simulink model "rfsoc4x2_ospfb_128"  (R2021a)
settings: Solver=VariableStepAuto  StartTime=0.0  StopTime=2048  RelTol=1e-3
undefined symbols (not defined in the file): pfb_coeff_gen_calc
libraries: xbsIndex_r4 x37092, casper_library_delays x737, casper_library_misc x68, xps_library x1
(part 157 of 339)

== system rfsoc4x2_ospfb_128/fft_wideband_real1/fft_unscrambler/reorder ==
  sync : Inport
  en : Inport  Port=2
  din0 : Inport  Port=3
  din1 : Inport  Port=4
  din2 : Inport  Port=5
  din3 : Inport  Port=6
  din4 : Inport  Port=7
  din5 : Inport  Port=8
  din6 : Inport  Port=9
  din7 : Inport  Port=10
  Counter : xbsIndex_r4/Counter  cnt_type=Free Running  cnt_to=Inf  operation=Up  start_count=0  cnt_by_val=1  arith_type=Unsigned  n_bits=4  bin_pt=0  load_pin=off  rst=on  en=on  explicit_period=on  period=1  use_behavioral_HDL=on  implementation=Fabric  dbl_ovrd=off  block_type=counter
  addr_expand : Subsystem  AncestorBlock=casper_library_flow_control/bus_expand  mask(bus_expand){mode=divisions of equal size, outputNum=8, outputWidth=4, outputBinaryPt=0, outputArithmeticType=0, show_format=off, outputToWorkspace=off, variablePrefix=out, outputToModelAsWell=on}
      mask prompts: outputNum "Number of outputs:"; outputWidth "Output width:"; outputBinaryPt "Output binary point position:"; outputArithmeticType "Output arithmetic type (ufix=0, fix=1, bool=2):"; show_format "Print format string?"; outputToWorkspace "Output to workspace?"; variablePrefix "Variable name prefix:"; outputToModelAsWell "Output to model as well?"
      mask help:
      | Expands a 'bus' made using a bus_create or Xilinx
      | concat block.
      | The input will be divided into the specified number
      | of outputs with the specified arithmetic types.
      | Divisions are made from most significant bit.
      mask init: same as rfsoc4x2_ospfb_128/bus_expand1
      settings: AttributesFormatString=8 outputs
      mask TypeOptions mode: divisions of equal size | divisions of arbitrary size
      mask Callback mode: %bus_expand_callback();
      mask Callback outputWidth: %bus_expand_callback();
      mask Callback outputToWorkspace: %bus_expand_callback();
  addr_replicate : Subsystem  AncestorBlock=casper_library_bus/bus_replicate  mask(bus_replicate){replication=8, csp_latency=3, misc=off, implementation=core}
      mask prompts: replication "replication factor"; csp_latency "latency"; misc "misc support"; implementation "delay implementation"
      mask help: Output bus formed by replicating input bus a number of times
      mask init:
      | bus_replicate_init(gcb, ...
      |     'replication', replication, ...
      |     'csp_latency', csp_latency, ...
      |     'implementation', implementation, ...
      |     'misc', misc);
      mask TypeOptions implementation: core | behavioral
  blank : xbsIndex_r4/Constant  const=0  gui_display_data_type=Fixed-point  arith_type=Unsigned  n_bits=4  bin_pt=0  preci_type=Single  exp_width=8  frac_width=24  explicit_period=on  period=1  equ=P=C  opselect=C  inp2=PCIN>>17  opr=+  inp1=P  carry=CIN  dbl_ovrd=off  block_type=constant
  buf0 : Subsystem  AncestorBlock=casper_library_bus/bus_single_port_ram  mask(bus_single_port_ram){n_bits=[[repmat(64, 1, 0)], 36], bin_pts=[zeros(1, 1)], init_vector=[zeros(16,1)], max_fanout=1, mem_type=Block RAM, bram_optimization=Speed, async=off, misc=off, bram_latency=3, fan_latency=0, addr_register=on, addr_implementation=core, din_register=on, din_implementation=behavioral, we_register=on, we_implementation=core, en_register=off, en_implementation=behavioral}
      mask prompts: n_bits "data word bit widths"; bin_pts "data word binary points"; init_vector "initial value vector"; max_fanout "limit fanout to ?"; mem_type "memory type"; bram_optimization "memory optimization"; async "asynchronous"; misc "misc support"; bram_latency "bram latency"; fan_latency "input register latency"; addr_register "addr input register"; addr_implementation "addr register implementation"; din_register "din input register"; din_implementation "din register implementation"; we_register "we input register"; we_implementation "we register implementation"; en_register "en input register"; en_implementation "en register implementation"
      mask help: RAM for a bus allowing fanout control
      mask init: same as rfsoc4x2_ospfb_128/fft2/fft_unscrambler/reorder/buf0
      mask TypeOptions mem_type: Distributed memory | Block RAM
      mask TypeOptions bram_optimization: Area | Speed
      mask TypeOptions addr_implementation: core | behavioral
      mask TypeOptions din_implementation: core | behavioral
      mask TypeOptions we_implementation: core | behavioral
      mask TypeOptions en_implementation: core | behavioral
  buf1 : Subsystem  AncestorBlock=casper_library_bus/bus_single_port_ram  mask(bus_single_port_ram){n_bits=[[repmat(64, 1, 0)], 36], bin_pts=[zeros(1, 1)], init_vector=[zeros(16,1)], max_fanout=1, mem_type=Block RAM, bram_optimization=Speed, async=off, misc=off, bram_latency=3, fan_latency=0, addr_register=on, addr_implementation=core, din_register=on, din_implementation=behavioral, we_register=on, we_implementation=core, en_register=off, en_implementation=behavioral}
      mask prompts: n_bits "data word bit widths"; bin_pts "data word binary points"; init_vector "initial value vector"; max_fanout "limit fanout to ?"; mem_type "memory type"; bram_optimization "memory optimization"; async "asynchronous"; misc "misc support"; bram_latency "bram latency"; fan_latency "input register latency"; addr_register "addr input register"; addr_implementation "addr register implementation"; din_register "din input register"; din_implementation "din register implementation"; we_register "we input register"; we_implementation "we register implementation"; en_register "en input register"; en_implementation "en register implementation"
      mask help: RAM for a bus allowing fanout control
      mask init: same as rfsoc4x2_ospfb_128/fft2/fft_unscrambler/reorder/buf0
      mask TypeOptions mem_type: Distributed memory | Block RAM
      mask TypeOptions bram_optimization: Area | Speed
      mask TypeOptions addr_implementation: core | behavioral
      mask TypeOptions din_implementation: core | behavioral
      mask TypeOptions we_implementation: core | behavioral
      mask TypeOptions en_implementation: core | behavioral
  buf2 : Subsystem  AncestorBlock=casper_library_bus/bus_single_port_ram  mask(bus_single_port_ram){n_bits=[[repmat(64, 1, 0)], 36], bin_pts=[zeros(1, 1)], init_vector=[zeros(16,1)], max_fanout=1, mem_type=Block RAM, bram_optimization=Speed, async=off, misc=off, bram_latency=3, fan_latency=0, addr_register=on, addr_implementation=core, din_register=on, din_implementation=behavioral, we_register=on, we_implementation=core, en_register=off, en_implementation=behavioral}
      mask prompts: n_bits "data word bit widths"; bin_pts "data word binary points"; init_vector "initial value vector"; max_fanout "limit fanout to ?"; mem_type "memory type"; bram_optimization "memory optimization"; async "asynchronous"; misc "misc support"; bram_latency "bram latency"; fan_latency "input register latency"; addr_register "addr input register"; addr_implementation "addr register implementation"; din_register "din input register"; din_implementation "din register implementation"; we_register "we input register"; we_implementation "we register implementation"; en_register "en input register"; en_implementation "en register implementation"
      mask help: RAM for a bus allowing fanout control
      mask init: same as rfsoc4x2_ospfb_128/fft2/fft_unscrambler/reorder/buf0
      mask TypeOptions mem_type: Distributed memory | Block RAM
      mask TypeOptions bram_optimization: Area | Speed
      mask TypeOptions addr_implementation: core | behavioral
      mask TypeOptions din_implementation: core | behavioral
      mask TypeOptions we_implementation: core | behavioral
      mask TypeOptions en_implementation: core | behavioral
  buf3 : Subsystem  AncestorBlock=casper_library_bus/bus_single_port_ram  mask(bus_single_port_ram){n_bits=[[repmat(64, 1, 0)], 36], bin_pts=[zeros(1, 1)], init_vector=[zeros(16,1)], max_fanout=1, mem_type=Block RAM, bram_optimization=Speed, async=off, misc=off, bram_latency=3, fan_latency=0, addr_register=on, addr_implementation=core, din_register=on, din_implementation=behavioral, we_register=on, we_implementation=core, en_register=off, en_implementation=behavioral}
      mask prompts: n_bits "data word bit widths"; bin_pts "data word binary points"; init_vector "initial value vector"; max_fanout "limit fanout to ?"; mem_type "memory type"; bram_optimization "memory optimization"; async "asynchronous"; misc "misc support"; bram_latency "bram latency"; fan_latency "input register latency"; addr_register "addr input register"; addr_implementation "addr register implementation"; din_register "din input register"; din_implementation "din register implementation"; we_register "we input register"; we_implementation "we register implementation"; en_register "en input register"; en_implementation "en register implementation"
      mask help: RAM for a bus allowing fanout control
      mask init: same as rfsoc4x2_ospfb_128/fft2/fft_unscrambler/reorder/buf0
      mask TypeOptions mem_type: Distributed memory | Block RAM
      mask TypeOptions bram_optimization: Area | Speed
      mask TypeOptions addr_implementation: core | behavioral
      mask TypeOptions din_implementation: core | behavioral
      mask TypeOptions we_implementation: core | behavioral
      mask TypeOptions en_implementation: core | behavioral
  buf4 : Subsystem  AncestorBlock=casper_library_bus/bus_single_port_ram  mask(bus_single_port_ram){n_bits=[[repmat(64, 1, 0)], 36], bin_pts=[zeros(1, 1)], init_vector=[zeros(16,1)], max_fanout=1, mem_type=Block RAM, bram_optimization=Speed, async=off, misc=off, bram_latency=3, fan_latency=0, addr_register=on, addr_implementation=core, din_register=on, din_implementation=behavioral, we_register=on, we_implementation=core, en_register=off, en_implementation=behavioral}
      mask prompts: n_bits "data word bit widths"; bin_pts "data word binary points"; init_vector "initial value vector"; max_fanout "limit fanout to ?"; mem_type "memory type"; bram_optimization "memory optimization"; async "asynchronous"; misc "misc support"; bram_latency "bram latency"; fan_latency "input register latency"; addr_register "addr input register"; addr_implementation "addr register implementation"; din_register "din input register"; din_implementation "din register implementation"; we_register "we input register"; we_implementation "we register implementation"; en_register "en input register"; en_implementation "en register implementation"
      mask help: RAM for a bus allowing fanout control
      mask init: same as rfsoc4x2_ospfb_128/fft2/fft_unscrambler/reorder/buf0
      mask TypeOptions mem_type: Distributed memory | Block RAM
      mask TypeOptions bram_optimization: Area | Speed
      mask TypeOptions addr_implementation: core | behavioral
      mask TypeOptions din_implementation: core | behavioral
      mask TypeOptions we_implementation: core | behavioral
      mask TypeOptions en_implementation: core | behavioral
  buf5 : Subsystem  AncestorBlock=casper_library_bus/bus_single_port_ram  mask(bus_single_port_ram){n_bits=[[repmat(64, 1, 0)], 36], bin_pts=[zeros(1, 1)], init_vector=[zeros(16,1)], max_fanout=1, mem_type=Block RAM, bram_optimization=Speed, async=off, misc=off, bram_latency=3, fan_latency=0, addr_register=on, addr_implementation=core, din_register=on, din_implementation=behavioral, we_register=on, we_implementation=core, en_register=off, en_implementation=behavioral}
      mask prompts: n_bits "data word bit widths"; bin_pts "data word binary points"; init_vector "initial value vector"; max_fanout "limit fanout to ?"; mem_type "memory type"; bram_optimization "memory optimization"; async "asynchronous"; misc "misc support"; bram_latency "bram latency"; fan_latency "input register latency"; addr_register "addr input register"; addr_implementation "addr register implementation"; din_register "din input register"; din_implementation "din register implementation"; we_register "we input register"; we_implementation "we register implementation"; en_register "en input register"; en_implementation "en register implementation"
      mask help: RAM for a bus allowing fanout control
      mask init: same as rfsoc4x2_ospfb_128/fft2/fft_unscrambler/reorder/buf0
      mask TypeOptions mem_type: Distributed memory | Block RAM
      mask TypeOptions bram_optimization: Area | Speed
      mask TypeOptions addr_implementation: core | behavioral
      mask TypeOptions din_implementation: core | behavioral
      mask TypeOptions we_implementation: core | behavioral
      mask TypeOptions en_implementation: core | behavioral
  buf6 : Subsystem  AncestorBlock=casper_library_bus/bus_single_port_ram  mask(bus_single_port_ram){n_bits=[[repmat(64, 1, 0)], 36], bin_pts=[zeros(1, 1)], init_vector=[zeros(16,1)], max_fanout=1, mem_type=Block RAM, bram_optimization=Speed, async=off, misc=off, bram_latency=3, fan_latency=0, addr_register=on, addr_implementation=core, din_register=on, din_implementation=behavioral, we_register=on, we_implementation=core, en_register=off, en_implementation=behavioral}
      mask prompts: n_bits "data word bit widths"; bin_pts "data word binary points"; init_vector "initial value vector"; max_fanout "limit fanout to ?"; mem_type "memory type"; bram_optimization "memory optimization"; async "asynchronous"; misc "misc support"; bram_latency "bram latency"; fan_latency "input register latency"; addr_register "addr input register"; addr_implementation "addr register implementation"; din_register "din input register"; din_implementation "din register implementation"; we_register "we input register"; we_implementation "we register implementation"; en_register "en input register"; en_implementation "en register implementation"
      mask help: RAM for a bus allowing fanout control
      mask init: same as rfsoc4x2_ospfb_128/fft2/fft_unscrambler/reorder/buf0
      mask TypeOptions mem_type: Distributed memory | Block RAM
      mask TypeOptions bram_optimization: Area | Speed
      mask TypeOptions addr_implementation: core | behavioral
      mask TypeOptions din_implementation: core | behavioral
      mask TypeOptions we_implementation: core | behavioral
      mask TypeOptions en_implementation: core | behavioral
  buf7 : Subsystem  AncestorBlock=casper_library_bus/bus_single_port_ram  mask(bus_single_port_ram){n_bits=[[repmat(64, 1, 0)], 36], bin_pts=[zeros(1, 1)], init_vector=[zeros(16,1)], max_fanout=1, mem_type=Block RAM, bram_optimization=Speed, async=off, misc=off, bram_latency=3, fan_latency=0, addr_register=on, addr_implementation=core, din_register=on, din_implementation=behavioral, we_register=on, we_implementation=core, en_register=off, en_implementation=behavioral}
      mask prompts: n_bits "data word bit widths"; bin_pts "data word binary points"; init_vector "initial value vector"; max_fanout "limit fanout to ?"; mem_type "memory type"; bram_optimization "memory optimization"; async "asynchronous"; misc "misc support"; bram_latency "bram latency"; fan_latency "input register latency"; addr_register "addr input register"; addr_implementation "addr register implementation"; din_register "din input register"; din_implementation "din register implementation"; we_register "we input register"; we_implementation "we register implementation"; en_register "en input register"; en_implementation "en register implementation"
      mask help: RAM for a bus allowing fanout control
      mask init: same as rfsoc4x2_ospfb_128/fft2/fft_unscrambler/reorder/buf0
      mask TypeOptions mem_type: Distributed memory | Block RAM
      mask TypeOptions bram_optimization: Area | Speed
      mask TypeOptions addr_implementation: core | behavioral
      mask TypeOptions din_implementation: core | behavioral
      mask TypeOptions we_implementation: core | behavioral
      mask TypeOptions en_implementation: core | behavioral
  current_map : Subsystem  AncestorBlock=casper_library_bus/bus_dual_port_ram  mask(bus_dual_port_ram){n_bits=4, bin_pts=0, init_vector=[0:15]', max_fanout=1, mem_type=Block RAM, bram_optimization=Speed, async_a=off, async_b=off, b_to_a_ratio_bits=0, misc=off, bram_latency=2, fan_latency=4, addra_register=on, addra_implementation=behavioral, dina_register=off, dina_implementation=behavioral, wea_register=on, wea_implementation=core, ena_register=off, ena_implementation=core, addrb_register=off, addrb_implementation=core, dinb_register=off, dinb_implementation=behavioral, web_register=off, web_implementation=behavioral, enb_register=off, enb_implementation=core}
      mask prompts: n_bits "data word bit widths"; bin_pts "data word binary points"; init_vector "initial value vector"; max_fanout "limit fanout to ?"; mem_type "memory type"; bram_optimization "memory optimization"; async_a "a asynchronous"; async_b "b asynchronous"; b_to_a_ratio_bits "b_to_a ratio bits"; misc "misc support"; bram_latency "bram latency"; fan_latency "input register latency"; addra_register "addra input register"; addra_implementation "addra register implementation"; dina_register "dina input register"; dina_implementation "dina register implementation"; wea_register "wea input register"; wea_implementation "wea register implementation"; ena_register "ena input register"; ena_implementation "ena register implementation"; addrb_register "addrb input register"; addrb_implementation "addrb register implementation"; dinb_register "dinb input register"; dinb_implementation "dinb register implementation"; web_register "web input register"; web_implementation "web register implementation"; enb_register "enb input register"; enb_implementation "enb register implementation"
      mask help: RAM for a bus allowing fanout control
      mask init:
      | bus_dual_port_ram_init(gcb, ...
      |     'n_bits', n_bits, ...
      |     'bin_pts', bin_pts, ...
      |     'init_vector', init_vector, ...
      |     'max_fanout', max_fanout, ...
      |     'mem_type', mem_type, ...
      |     'bram_optimization', bram_optimization, ...
      |     'async_a', async_a, ...
      |     'async_b', async_b, ...
      |     'b_to_a_ratio_bits', b_to_a_ratio_bits, ...
      |     'misc', misc, ...
      |     'bram_latency', bram_latency, ...
      |     'fan_latency', fan_latency, ...
      |     'addra_register', addra_register, ...
      |     'addra_implementation', addra_implementation, ...
      |     'dina_register', dina_register, ...
      |     'dina_implementation', dina_implementation, ...
      |     'wea_register', wea_register, ...
      |     'wea_implementation', wea_implementation, ...
      |     'ena_register', ena_register, ...
      |     'ena_implementation', ena_implementation, ...
      |     'addrb_register', addrb_register, ...
      |     'addrb_implementation', addrb_implementation, ...
      |     'dinb_register', dinb_register, ...
      |     'dinb_implementation', dinb_implementation, ...
      |     'web_register', web_register, ...
      |     'web_implementation', web_implementation, ...
      |     'enb_register', enb_register, ...
      |     'enb_implementation', enb_implementation);
      mask TypeOptions mem_type: Distributed memory | Block RAM
      mask TypeOptions bram_optimization: Area | Speed
      mask TypeOptions addra_implementation: core | behavioral
      mask TypeOptions dina_implementation: core | behavioral
      mask TypeOptions wea_implementation: core | behavioral
      mask TypeOptions ena_implementation: core | behavioral
      mask TypeOptions addrb_implementation: core | behavioral
      mask TypeOptions dinb_implementation: core | behavioral
      mask TypeOptions web_implementation: core | behavioral
      mask TypeOptions enb_implementation: core | behavioral
  daddr0 : xbsIndex_r4/Delay  rst=off  infoeditControl=Selection of Reset will increase slice count due to use of real FFs and instead of SRLs  en=off  latency=1  reg_retiming=on  dbl_ovrd=off  block_type=delay
  daddr1 : xbsIndex_r4/Delay  rst=off  infoeditControl=Selection of Reset will increase slice count due to use of real FFs and instead of SRLs  en=off  latency=2  reg_retiming=on  dbl_ovrd=off  block_type=delay
  delay_din{0..7} (8 alike) : xbsIndex_r4/Delay  rst=off  infoeditControl=Selection of Reset will increase slice count due to use of real FFs and instead of SRLs  en=off  latency=7  reg_retiming=on  dbl_ovrd=off  block_type=delay
  delay_valid : xbsIndex_r4/Delay  rst=off  infoeditControl=Selection of Reset will increase slice count due to use of real FFs and instead of SRLs  en=off  latency=3  reg_retiming=on  dbl_ovrd=off  block_type=delay
  delay_we0 : xbsIndex_r4/Delay  rst=off  infoeditControl=Selection of Reset will increase slice count due to use of real FFs and instead of SRLs  en=off  latency=7  reg_retiming=on  dbl_ovrd=off  block_type=delay
  delay_we1 : xbsIndex_r4/Delay  rst=off  infoeditControl=Selection of Reset will increase slice count due to use of real FFs and instead of SRLs  en=off  latency=7  reg_retiming=on  dbl_ovrd=off  block_type=delay
  delay_we2 : xbsIndex_r4/Delay  rst=off  infoeditControl=Selection of Reset will increase slice count due to use of real FFs and instead of SRLs  en=off  latency=4  reg_retiming=on  dbl_ovrd=off  block_type=delay
  den : xbsIndex_r4/Delay  rst=off  infoeditControl=Selection of Reset will increase slice count due to use of real FFs and instead of SRLs  en=off  latency=3  reg_retiming=on  dbl_ovrd=off  block_type=delay
  dmap_src : xbsIndex_r4/Delay  rst=off  infoeditControl=Selection of Reset will increase slice count due to use of real FFs and instead of SRLs  en=off  latency=2  reg_retiming=on  dbl_ovrd=off  block_type=delay
  dnew_map : xbsIndex_r4/Delay  rst=off  infoeditControl=Selection of Reset will increase slice count due to use of real FFs and instead of SRLs  en=off  latency=1  reg_retiming=on  dbl_ovrd=off  block_type=delay
  dsync : xbsIndex_r4/Delay  rst=off  infoeditControl=Selection of Reset will increase slice count due to use of real FFs and instead of SRLs  en=off  latency=1  reg_retiming=on  dbl_ovrd=off  block_type=delay
  edge_detect : Subsystem  AncestorBlock=casper_library_misc/edge_detect  mask(edge_detect){edge=Falling, polarity=Active High, x_in=[0 0.08 0.08 0.16 0.16 0.24 0.24 0.32 0.32 0.4], y_in=[-1 -1  1  1  1  1  1  1  1  1], x_out=[0.6 0.68 0.68 0.76 0.76 0.84 0.84 0.92 0.92 1], y_out=[-1 -1  1  1 -1 -1 -1 -1 -1 -1]}
      mask prompts: edge "Edge Type"; polarity "Output Polarity"; x_in "Input X Positions"; y_in "Input Y Positions"; x_out "Output X Positions"; y_out "Output Y Positions"
      mask help: Output is active for one-cycle after each edge of the specified type (i.e. rising, falling or both).
      mask init: same as rfsoc4x2_ospfb_128/edge_detect10
      settings: AttributesFormatString=|
      | falling edges
      | active high
      mask Help: Output is active for one-cycle after each edge of the specified type (i.e. rising, falling, or both).  Latency is zero.
      mask TypeOptions edge: Rising | Falling | Both
      mask TypeOptions polarity: Active High | Active Low
      mask Display:
      | plot(x_in_num,0.5+y_in_num*0.2);
      | plot(x_out_num,0.5+y_out_num*0.2);
  map_mod : xbsIndex_r4/ROM  depth=16  initVector=map  distributed_mem=Block RAM  rst=off  init_reg=0  en=off  latency=2  gui_display_data_type=Fixed-point  arith_type=Unsigned  n_bits=4  bin_pt=0  preci_type=Single  exp_width=8  frac_width=24  optimize=Speed  use_rpm=on  dbl_ovrd=off  simulation_type=fast_sim  block_type=sprom
  map_mux : xbsIndex_r4/Mux  inputs=2  en=off  latency=1  precision=Full  arith_type=Unsigned  n_bits=16  bin_pt=14  quantization=Truncate  overflow=Wrap  dbl_ovrd=off  block_type=mux
  map_src : xbsIndex_r4/Register  init=0  rst=on  en=on  dbl_ovrd=off  block_type=register
  msb : xbsIndex_r4/Slice  nbits=1  boolean_output=on  mode=Upper Bit Location + Width  bit1=0  base1=MSB of Input  bit0=0  base0=LSB of Input  dbl_ovrd=off  block_type=slice
  never : xbsIndex_r4/Constant  const=0  gui_display_data_type=Fixed-point  arith_type=Boolean  n_bits=16  bin_pt=14  preci_type=Single  exp_width=8  frac_width=24  explicit_period=on  period=1  equ=P=C  opselect=C  inp2=PCIN>>17  opr=+  inp1=P  carry=CIN  dbl_ovrd=off  block_type=constant
  or : xbsIndex_r4/Logical  logical_function=OR  inputs=2  en=off  latency=0  precision=Full  arith_type=Unsigned  n_bits=16  bin_pt=0  align_bp=on  dbl_ovrd=off  block_type=logical
  post_sync_delay : xbsIndex_r4/Delay  rst=off  infoeditControl=Selection of Reset will increase slice count due to use of real FFs and instead of SRLs  en=off  latency=3  reg_retiming=on  dbl_ovrd=off  block_type=delay
  pre_sync_delay : xbsIndex_r4/Delay  rst=off  infoeditControl=Selection of Reset will increase slice count due to use of real FFs and instead of SRLs  en=off  latency=7  reg_retiming=on  dbl_ovrd=off  block_type=delay
  sync_delay_en : casper_library_delays/sync_delay_en  DelayLen=16
      settings: SourceProductName=CASPER DSP Blockset
  term : Terminator
  we_expand : Subsystem  AncestorBlock=casper_library_flow_control/bus_expand  mask(bus_expand){mode=divisions of equal size, outputNum=8, outputWidth=1, outputBinaryPt=0, outputArithmeticType=2, show_format=off, outputToWorkspace=off, variablePrefix=out, outputToModelAsWell=on}
      mask prompts: outputNum "Number of outputs:"; outputWidth "Output width:"; outputBinaryPt "Output binary point position:"; outputArithmeticType "Output arithmetic type (ufix=0, fix=1, bool=2):"; show_format "Print format string?"; outputToWorkspace "Output to workspace?"; variablePrefix "Variable name prefix:"; outputToModelAsWell "Output to model as well?"
      mask help:
      | Expands a 'bus' made using a bus_create or Xilinx
      | concat block.
      | The input will be divided into the specified number
      | of outputs with the specified arithmetic types.
      | Divisions are made from most significant bit.
      mask init: same as rfsoc4x2_ospfb_128/bus_expand1
      settings: AttributesFormatString=8 outputs
      mask TypeOptions mode: divisions of equal size | divisions of arbitrary size
      mask Callback mode: %bus_expand_callback();
      mask Callback outputWidth: %bus_expand_callback();
      mask Callback outputToWorkspace: %bus_expand_callback();
  we_replicate : Subsystem  AncestorBlock=casper_library_bus/bus_replicate  mask(bus_replicate){replication=8, csp_latency=3, misc=off, implementation=core}
      mask prompts: replication "replication factor"; csp_latency "latency"; misc "misc support"; implementation "delay implementation"
      mask help: Output bus formed by replicating input bus a number of times
      mask init:
      | bus_replicate_init(gcb, ...
      |     'replication', replication, ...
      |     'csp_latency', csp_latency, ...
      |     'implementation', implementation, ...
      |     'misc', misc);
      mask TypeOptions implementation: core | behavioral
  sync_out : Outport
  valid : Outport  Port=2
  dout0 : Outport  Port=3
  dout1 : Outport  Port=4
  dout2 : Outport  Port=5
  dout3 : Outport  Port=6
  dout4 : Outport  Port=7
  dout5 : Outport  Port=8
  dout6 : Outport  Port=9
  dout7 : Outport  Port=10
  wires:
  dnew_map/1 -> current_map/2(dina)
  map_mod/1 -> dnew_map/1
  daddr1/1 -> current_map/1(addra), map_mux/2
  den/1 -> current_map/3(wea)
  never/1 -> current_map/6(web)
  blank/1 -> current_map/5(dinb)
  current_map/1(A) -> term/1
  current_map/2(B) -> map_mux/3
  daddr0/1 -> daddr1/1, current_map/4(addrb)
  map_mux/1 -> map_mod/1, addr_replicate/1(in)
  dmap_src/1 -> map_mux/1
  map_src/1 -> dmap_src/1
  dsync/1 -> map_src/2
  edge_detect/1(out) -> map_src/3, map_src/1
  msb/1 -> edge_detect/1(in)
  Counter/1 -> daddr0/1, msb/1
  buf7/1(dout) -> dout7/1
  delay_din7/1 -> buf7/2(din)
  addr_expand/8(lsb_out1) -> buf7/1(addr)
  we_expand/8(lsb_out1) -> buf7/3(we)
  buf6/1(dout) -> dout6/1
  delay_din6/1 -> buf6/2(din)
  addr_expand/7(out2) -> buf6/1(addr)
  we_expand/7(out2) -> buf6/3(we)
  buf5/1(dout) -> dout5/1
  delay_din5/1 -> buf5/2(din)
  addr_expand/6(out3) -> buf5/1(addr)
  we_expand/6(out3) -> buf5/3(we)
  buf4/1(dout) -> dout4/1
  delay_din4/1 -> buf4/2(din)
  addr_expand/5(out4) -> buf4/1(addr)
  we_expand/5(out4) -> buf4/3(we)
  buf3/1(dout) -> dout3/1
  delay_din3/1 -> buf3/2(din)
  addr_expand/4(out5) -> buf3/1(addr)
  we_expand/4(out5) -> buf3/3(we)
  buf2/1(dout) -> dout2/1
  delay_din2/1 -> buf2/2(din)
  addr_expand/3(out6) -> buf2/1(addr)
  we_expand/3(out6) -> buf2/3(we)
  buf1/1(dout) -> dout1/1
  delay_din1/1 -> buf1/2(din)
  addr_expand/2(out7) -> buf1/1(addr)
  we_expand/2(out7) -> buf1/3(we)
  buf0/1(dout) -> dout0/1
  delay_din0/1 -> buf0/2(din)
  addr_expand/1(msb_out8) -> buf0/1(addr)
  we_expand/1(msb_out8) -> buf0/3(we)
  addr_replicate/1(out) -> addr_expand/1(bus_in)
  din7/1 -> delay_din7/1
  din6/1 -> delay_din6/1
  din5/1 -> delay_din5/1
  din4/1 -> delay_din4/1
  din3/1 -> delay_din3/1
  din2/1 -> delay_din2/1
  din1/1 -> delay_din1/1
  din0/1 -> delay_din0/1
  post_sync_delay/1 -> sync_out/1
  sync_delay_en/1 -> post_sync_delay/1
  or/1 -> sync_delay_en/2
  pre_sync_delay/1 -> sync_delay_en/1, or/1
  delay_we0/1 -> or/2
  sync/1 -> dsync/1, Counter/1, pre_sync_delay/1
  we_replicate/1(out) -> we_expand/1(bus_in)
  delay_we2/1 -> we_replicate/1(in)
  delay_valid/1 -> valid/1
  delay_we1/1 -> delay_valid/1
  en/1 -> den/1, Counter/2, delay_we2/1, delay_we1/1, delay_we0/1

== system rfsoc4x2_ospfb_128/fft_wideband_real1/fft_unscrambler/square_transposer ==
  sync : Inport
  in0 : Inport  Port=2
  in1 : Inport  Port=3
  in2 : Inport  Port=4
  in3 : Inport  Port=5
  in4 : Inport  Port=6
  in5 : Inport  Port=7
  in6 : Inport  Port=8
  in7 : Inport  Port=9
  barrel_switcher : Subsystem  AncestorBlock=casper_library_reorder/barrel_switcher  mask(barrel_switcher){n_inputs=3, async=off}
      mask prompts: n_inputs "Number of Inputs: (2^?)"; async "Asynchronous operation"
      mask help:
      | Shifts input to right by amount specified on sel,
      | wrapping around into higher order bits.
      mask init:
      | barrel_switcher_init(gcb,...
      |     'n_inputs', n_inputs, ...
      |     'async', async);
      mask Help: eval('xlWeb(''http://casper.berkeley.edu/wiki/Barrel_switcher'')')
  counter : xbsIndex_r4/Counter  cnt_type=Free Running  cnt_to=Inf  operation=Down  start_count=0  cnt_by_val=1  arith_type=Unsigned  n_bits=n_inputs  bin_pt=0  load_pin=off  rst=on  en=off  explicit_period=on  period=1  use_behavioral_HDL=off  implementation=Fabric  dbl_ovrd=off  block_type=counter
  db0 : Subsystem  AncestorBlock=casper_library_delays/delay_slr  mask(delay_slr){DelayLen=7, async=off}
      mask prompts: DelayLen "Delay by:"; async "asynchronous operation"
      mask help: A delay block that uses slices (SLR16s) for its storage.
      mask init:
      | delay_slr_init(gcb, ...
      |     'DelayLen', DelayLen, ...
      |     'async', async);
  db1 : Subsystem  AncestorBlock=casper_library_delays/delay_slr  mask(delay_slr){DelayLen=6, async=off}
      mask prompts: DelayLen "Delay by:"; async "asynchronous operation"
      mask help: A delay block that uses slices (SLR16s) for its storage.
      mask init:
      | delay_slr_init(gcb, ...
      |     'DelayLen', DelayLen, ...
      |     'async', async);
  db2 : Subsystem  AncestorBlock=casper_library_delays/delay_slr  mask(delay_slr){DelayLen=5, async=off}
      mask prompts: DelayLen "Delay by:"; async "asynchronous operation"
      mask help: A delay block that uses slices (SLR16s) for its storage.
      mask init:
      | delay_slr_init(gcb, ...
      |     'DelayLen', DelayLen, ...
      |     'async', async);
  db3 : Subsystem  AncestorBlock=casper_library_delays/delay_slr  mask(delay_slr){DelayLen=4, async=off}
      mask prompts: DelayLen "Delay by:"; async "asynchronous operation"
      mask help: A delay block that uses slices (SLR16s) for its storage.
      mask init:
      | delay_slr_init(gcb, ...
      |     'DelayLen', DelayLen, ...
      |     'async', async);
  db4 : Subsystem  AncestorBlock=casper_library_delays/delay_slr  mask(delay_slr){DelayLen=3, async=off}
      mask prompts: DelayLen "Delay by:"; async "asynchronous operation"
      mask help: A delay block that uses slices (SLR16s) for its storage.
      mask init:
      | delay_slr_init(gcb, ...
      |     'DelayLen', DelayLen, ...
      |     'async', async);
  db5 : Subsystem  AncestorBlock=casper_library_delays/delay_slr  mask(delay_slr){DelayLen=2, async=off}
      mask prompts: DelayLen "Delay by:"; async "asynchronous operation"
      mask help: A delay block that uses slices (SLR16s) for its storage.
      mask init:
      | delay_slr_init(gcb, ...
      |     'DelayLen', DelayLen, ...
      |     'async', async);
  db6 : Subsystem  AncestorBlock=casper_library_delays/delay_slr  mask(delay_slr){DelayLen=1, async=off}
      mask prompts: DelayLen "Delay by:"; async "asynchronous operation"
      mask help: A delay block that uses slices (SLR16s) for its storage.
      mask init:
      | delay_slr_init(gcb, ...
      |     'DelayLen', DelayLen, ...
      |     'async', async);
  df1 : Subsystem  AncestorBlock=casper_library_delays/delay_slr  mask(delay_slr){DelayLen=1, async=off}
      mask prompts: DelayLen "Delay by:"; async "asynchronous operation"
      mask help: A delay block that uses slices (SLR16s) for its storage.
      mask init:
      | delay_slr_init(gcb, ...
      |     'DelayLen', DelayLen, ...
      |     'async', async);
  df2 : Subsystem  AncestorBlock=casper_library_delays/delay_slr  mask(delay_slr){DelayLen=2, async=off}
      mask prompts: DelayLen "Delay by:"; async "asynchronous operation"
      mask help: A delay block that uses slices (SLR16s) for its storage.
      mask init:
      | delay_slr_init(gcb, ...
      |     'DelayLen', DelayLen, ...
      |     'async', async);
  df3 : Subsystem  AncestorBlock=casper_library_delays/delay_slr  mask(delay_slr){DelayLen=3, async=off}
      mask prompts: DelayLen "Delay by:"; async "asynchronous operation"
      mask help: A delay block that uses slices (SLR16s) for its storage.
      mask init:
      | delay_slr_init(gcb, ...
      |     'DelayLen', DelayLen, ...
      |     'async', async);
  df4 : Subsystem  AncestorBlock=casper_library_delays/delay_slr  mask(delay_slr){DelayLen=4, async=off}
      mask prompts: DelayLen "Delay by:"; async "asynchronous operation"
      mask help: A delay block that uses slices (SLR16s) for its storage.
      mask init:
      | delay_slr_init(gcb, ...
      |     'DelayLen', DelayLen, ...
      |     'async', async);
  df5 : Subsystem  AncestorBlock=casper_library_delays/delay_slr  mask(delay_slr){DelayLen=5, async=off}
      mask prompts: DelayLen "Delay by:"; async "asynchronous operation"
      mask help: A delay block that uses slices (SLR16s) for its storage.
      mask init:
      | delay_slr_init(gcb, ...
      |     'DelayLen', DelayLen, ...
      |     'async', async);
  df6 : Subsystem  AncestorBlock=casper_library_delays/delay_slr  mask(delay_slr){DelayLen=6, async=off}
      mask prompts: DelayLen "Delay by:"; async "asynchronous operation"
      mask help: A delay block that uses slices (SLR16s) for its storage.
      mask init:
      | delay_slr_init(gcb, ...
      |     'DelayLen', DelayLen, ...
      |     'async', async);
  df7 : Subsystem  AncestorBlock=casper_library_delays/delay_slr  mask(delay_slr){DelayLen=7, async=off}
      mask prompts: DelayLen "Delay by:"; async "asynchronous operation"
      mask help: A delay block that uses slices (SLR16s) for its storage.
      mask init:
      | delay_slr_init(gcb, ...
      |     'DelayLen', DelayLen, ...
      |     'async', async);
  dsync : Subsystem  AncestorBlock=casper_library_delays/delay_slr  mask(delay_slr){DelayLen=7, async=off}
      mask prompts: DelayLen "Delay by:"; async "asynchronous operation"
      mask help: A delay block that uses slices (SLR16s) for its storage.
      mask init:
      | delay_slr_init(gcb, ...
      |     'DelayLen', DelayLen, ...
      |     'async', async);
  sync_out : Outport
  out0 : Outport  Port=2
  out1 : Outport  Port=3
  out2 : Outport  Port=4
  out3 : Outport  Port=5
  out4 : Outport  Port=6
  out5 : Outport  Port=7
  out6 : Outport  Port=8
  out7 : Outport  Port=9
  wires:
  barrel_switcher/9(Out8) -> out7/1
  df7/1(dout) -> barrel_switcher/4(In2)
  in7/1 -> df7/1(din)
  db6/1(dout) -> out6/1
  barrel_switcher/8(Out7) -> db6/1(din)
  df6/1(dout) -> barrel_switcher/5(In3)
  in6/1 -> df6/1(din)
  db5/1(dout) -> out5/1
  barrel_switcher/7(Out6) -> db5/1(din)
  df5/1(dout) -> barrel_switcher/6(In4)
  in5/1 -> df5/1(din)
  db4/1(dout) -> out4/1
  barrel_switcher/6(Out5) -> db4/1(din)
  df4/1(dout) -> barrel_switcher/7(In5)
  in4/1 -> df4/1(din)
  db3/1(dout) -> out3/1
  barrel_switcher/5(Out4) -> db3/1(din)
  df3/1(dout) -> barrel_switcher/8(In6)
  in3/1 -> df3/1(din)
  db2/1(dout) -> out2/1
  barrel_switcher/4(Out3) -> db2/1(din)
  df2/1(dout) -> barrel_switcher/9(In7)
  in2/1 -> df2/1(din)
  db1/1(dout) -> out1/1
  barrel_switcher/3(Out2) -> db1/1(din)
  df1/1(dout) -> barrel_switcher/10(In8)
  in1/1 -> df1/1(din)
  db0/1(dout) -> out0/1
  barrel_switcher/2(Out1) -> db0/1(din)
  in0/1 -> barrel_switcher/3(In1)
  barrel_switcher/1(sync_out) -> dsync/1(din)
  counter/1 -> barrel_switcher/1(sel)
  dsync/1(dout) -> sync_out/1
  sync/1 -> barrel_switcher/2(sync_in), counter/1

== system rfsoc4x2_ospfb_128/pfb_fir_real10/pol1_in1_first_tap/delay_bram ==
  din : Inport
  constant : xbsIndex_r4/Constant  const=1  gui_display_data_type=Fixed-point  arith_type=Boolean  n_bits=16  bin_pt=14  preci_type=Single  exp_width=8  frac_width=24  explicit_period=on  period=1  equ=P=C  opselect=C  inp2=PCIN>>17  opr=+  inp1=P  carry=CIN  dbl_ovrd=off  block_type=constant
  counter : xbsIndex_r4/Counter  cnt_type=Count Limited  cnt_to=DelayLen - bram_latency - 1  operation=Up  start_count=0  cnt_by_val=1  arith_type=Unsigned  n_bits=4  bin_pt=0  load_pin=off  rst=off  en=off  explicit_period=on  period=1  use_behavioral_HDL=on  implementation=Fabric  use_rpm=off  dbl_ovrd=off  block_type=counter
  ram : xbsIndex_r4/Single Port RAM  depth=16  initVector=0  distributed_mem=Block RAM  write_mode=Read Before Write  rst=off  init_reg=0  en=off  optimize_latency=off  latency=bram_latency  optimize=Area  dbl_ovrd=off  simulation_type=fast_sim  block_type=spram
  dout : Outport  VectorParamsAs1DForOutWhenUnconnected=off
  wires:
  ram/1 -> dout/1
  constant/1 -> ram/3
  din/1 -> ram/2
  counter/1 -> ram/1

== system rfsoc4x2_ospfb_128/pfb_fir_real10/pol1_in1_first_tap1/delay_bram ==
  din : Inport
  constant : xbsIndex_r4/Constant  const=1  gui_display_data_type=Fixed-point  arith_type=Boolean  n_bits=16  bin_pt=14  preci_type=Single  exp_width=8  frac_width=24  explicit_period=on  period=1  equ=P=C  opselect=C  inp2=PCIN>>17  opr=+  inp1=P  carry=CIN  dbl_ovrd=off  block_type=constant
  counter : xbsIndex_r4/Counter  cnt_type=Count Limited  cnt_to=DelayLen - bram_latency - 1  operation=Up  start_count=0  cnt_by_val=1  arith_type=Unsigned  n_bits=4  bin_pt=0  load_pin=off  rst=off  en=off  explicit_period=on  period=1  use_behavioral_HDL=on  implementation=Fabric  use_rpm=off  dbl_ovrd=off  block_type=counter
  ram : xbsIndex_r4/Single Port RAM  depth=16  initVector=0  distributed_mem=Block RAM  write_mode=Read Before Write  rst=off  init_reg=0  en=off  optimize_latency=off  latency=bram_latency  optimize=Area  dbl_ovrd=off  simulation_type=fast_sim  block_type=spram
  dout : Outport  VectorParamsAs1DForOutWhenUnconnected=off
  wires:
  counter/1 -> ram/1
  din/1 -> ram/2
  constant/1 -> ram/3
  ram/1 -> dout/1

== system rfsoc4x2_ospfb_128/pfb_fir_real10/pol1_in1_first_tap10/delay_bram ==
  din : Inport
  constant : xbsIndex_r4/Constant  const=1  gui_display_data_type=Fixed-point  arith_type=Boolean  n_bits=16  bin_pt=14  preci_type=Single  exp_width=8  frac_width=24  explicit_period=on  period=1  equ=P=C  opselect=C  inp2=PCIN>>17  opr=+  inp1=P  carry=CIN  dbl_ovrd=off  block_type=constant
  counter : xbsIndex_r4/Counter  cnt_type=Count Limited  cnt_to=DelayLen - bram_latency - 1  operation=Up  start_count=0  cnt_by_val=1  arith_type=Unsigned  n_bits=4  bin_pt=0  load_pin=off  rst=off  en=off  explicit_period=on  period=1  use_behavioral_HDL=on  implementation=Fabric  use_rpm=off  dbl_ovrd=off  block_type=counter
  ram : xbsIndex_r4/Single Port RAM  depth=16  initVector=0  distributed_mem=Block RAM  write_mode=Read Before Write  rst=off  init_reg=0  en=off  optimize_latency=off  latency=bram_latency  optimize=Area  dbl_ovrd=off  simulation_type=fast_sim  block_type=spram
  dout : Outport  VectorParamsAs1DForOutWhenUnconnected=off
  wires:
  counter/1 -> ram/1
  din/1 -> ram/2
  constant/1 -> ram/3
  ram/1 -> dout/1

== system rfsoc4x2_ospfb_128/pfb_fir_real10/pol1_in1_first_tap11/delay_bram ==
  din : Inport
  constant : xbsIndex_r4/Constant  const=1  gui_display_data_type=Fixed-point  arith_type=Boolean  n_bits=16  bin_pt=14  preci_type=Single  exp_width=8  frac_width=24  explicit_period=on  period=1  equ=P=C  opselect=C  inp2=PCIN>>17  opr=+  inp1=P  carry=CIN  dbl_ovrd=off  block_type=constant
  counter : xbsIndex_r4/Counter  cnt_type=Count Limited  cnt_to=DelayLen - bram_latency - 1  operation=Up  start_count=0  cnt_by_val=1  arith_type=Unsigned  n_bits=4  bin_pt=0  load_pin=off  rst=off  en=off  explicit_period=on  period=1  use_behavioral_HDL=on  implementation=Fabric  use_rpm=off  dbl_ovrd=off  block_type=counter
  ram : xbsIndex_r4/Single Port RAM  depth=16  initVector=0  distributed_mem=Block RAM  write_mode=Read Before Write  rst=off  init_reg=0  en=off  optimize_latency=off  latency=bram_latency  optimize=Area  dbl_ovrd=off  simulation_type=fast_sim  block_type=spram
  dout : Outport  VectorParamsAs1DForOutWhenUnconnected=off
  wires:
  counter/1 -> ram/1
  din/1 -> ram/2
  constant/1 -> ram/3
  ram/1 -> dout/1

== system rfsoc4x2_ospfb_128/pfb_fir_real10/pol1_in1_first_tap12/delay_bram ==
  din : Inport
  constant : xbsIndex_r4/Constant  const=1  gui_display_data_type=Fixed-point  arith_type=Boolean  n_bits=16  bin_pt=14  preci_type=Single  exp_width=8  frac_width=24  explicit_period=on  period=1  equ=P=C  opselect=C  inp2=PCIN>>17  opr=+  inp1=P  carry=CIN  dbl_ovrd=off  block_type=constant
  counter : xbsIndex_r4/Counter  cnt_type=Count Limited  cnt_to=DelayLen - bram_latency - 1  operation=Up  start_count=0  cnt_by_val=1  arith_type=Unsigned  n_bits=4  bin_pt=0  load_pin=off  rst=off  en=off  explicit_period=on  period=1  use_behavioral_HDL=on  implementation=Fabric  use_rpm=off  dbl_ovrd=off  block_type=counter
  ram : xbsIndex_r4/Single Port RAM  depth=16  initVector=0  distributed_mem=Block RAM  write_mode=Read Before Write  rst=off  init_reg=0  en=off  optimize_latency=off  latency=bram_latency  optimize=Area  dbl_ovrd=off  simulation_type=fast_sim  block_type=spram
  dout : Outport  VectorParamsAs1DForOutWhenUnconnected=off
  wires:
  counter/1 -> ram/1
  din/1 -> ram/2
  constant/1 -> ram/3
  ram/1 -> dout/1

== system rfsoc4x2_ospfb_128/pfb_fir_real10/pol1_in1_first_tap13/delay_bram ==
  din : Inport
  constant : xbsIndex_r4/Constant  const=1  gui_display_data_type=Fixed-point  arith_type=Boolean  n_bits=16  bin_pt=14  preci_type=Single  exp_width=8  frac_width=24  explicit_period=on  period=1  equ=P=C  opselect=C  inp2=PCIN>>17  opr=+  inp1=P  carry=CIN  dbl_ovrd=off  block_type=constant
  counter : xbsIndex_r4/Counter  cnt_type=Count Limited  cnt_to=DelayLen - bram_latency - 1  operation=Up  start_count=0  cnt_by_val=1  arith_type=Unsigned  n_bits=4  bin_pt=0  load_pin=off  rst=off  en=off  explicit_period=on  period=1  use_behavioral_HDL=on  implementation=Fabric  use_rpm=off  dbl_ovrd=off  block_type=counter
  ram : xbsIndex_r4/Single Port RAM  depth=16  initVector=0  distributed_mem=Block RAM  write_mode=Read Before Write  rst=off  init_reg=0  en=off  optimize_latency=off  latency=bram_latency  optimize=Area  dbl_ovrd=off  simulation_type=fast_sim  block_type=spram
  dout : Outport  VectorParamsAs1DForOutWhenUnconnected=off
  wires:
  counter/1 -> ram/1
  din/1 -> ram/2
  constant/1 -> ram/3
  ram/1 -> dout/1

== system rfsoc4x2_ospfb_128/pfb_fir_real10/pol1_in1_first_tap14/delay_bram ==
  din : Inport
  constant : xbsIndex_r4/Constant  const=1  gui_display_data_type=Fixed-point  arith_type=Boolean  n_bits=16  bin_pt=14  preci_type=Single  exp_width=8  frac_width=24  explicit_period=on  period=1  equ=P=C  opselect=C  inp2=PCIN>>17  opr=+  inp1=P  carry=CIN  dbl_ovrd=off  block_type=constant
  counter : xbsIndex_r4/Counter  cnt_type=Count Limited  cnt_to=DelayLen - bram_latency - 1  operation=Up  start_count=0  cnt_by_val=1  arith_type=Unsigned  n_bits=4  bin_pt=0  load_pin=off  rst=off  en=off  explicit_period=on  period=1  use_behavioral_HDL=on  implementation=Fabric  use_rpm=off  dbl_ovrd=off  block_type=counter
  ram : xbsIndex_r4/Single Port RAM  depth=16  initVector=0  distributed_mem=Block RAM  write_mode=Read Before Write  rst=off  init_reg=0  en=off  optimize_latency=off  latency=bram_latency  optimize=Area  dbl_ovrd=off  simulation_type=fast_sim  block_type=spram
  dout : Outport  VectorParamsAs1DForOutWhenUnconnected=off
  wires:
  counter/1 -> ram/1
  din/1 -> ram/2
  constant/1 -> ram/3
  ram/1 -> dout/1

== system rfsoc4x2_ospfb_128/pfb_fir_real10/pol1_in1_first_tap15/delay_bram ==
  din : Inport
  constant : xbsIndex_r4/Constant  const=1  gui_display_data_type=Fixed-point  arith_type=Boolean  n_bits=16  bin_pt=14  preci_type=Single  exp_width=8  frac_width=24  explicit_period=on  period=1  equ=P=C  opselect=C  inp2=PCIN>>17  opr=+  inp1=P  carry=CIN  dbl_ovrd=off  block_type=constant
  counter : xbsIndex_r4/Counter  cnt_type=Count Limited  cnt_to=DelayLen - bram_latency - 1  operation=Up  start_count=0  cnt_by_val=1  arith_type=Unsigned  n_bits=4  bin_pt=0  load_pin=off  rst=off  en=off  explicit_period=on  period=1  use_behavioral_HDL=on  implementation=Fabric  use_rpm=off  dbl_ovrd=off  block_type=counter
  ram : xbsIndex_r4/Single Port RAM  depth=16  initVector=0  distributed_mem=Block RAM  write_mode=Read Before Write  rst=off  init_reg=0  en=off  optimize_latency=off  latency=bram_latency  optimize=Area  dbl_ovrd=off  simulation_type=fast_sim  block_type=spram
  dout : Outport  VectorParamsAs1DForOutWhenUnconnected=off
  wires:
  counter/1 -> ram/1
  din/1 -> ram/2
  constant/1 -> ram/3
  ram/1 -> dout/1

== system rfsoc4x2_ospfb_128/pfb_fir_real10/pol1_in1_first_tap2/delay_bram ==
  din : Inport
  constant : xbsIndex_r4/Constant  const=1  gui_display_data_type=Fixed-point  arith_type=Boolean  n_bits=16  bin_pt=14  preci_type=Single  exp_width=8  frac_width=24  explicit_period=on  period=1  equ=P=C  opselect=C  inp2=PCIN>>17  opr=+  inp1=P  carry=CIN  dbl_ovrd=off  block_type=constant
  counter : xbsIndex_r4/Counter  cnt_type=Count Limited  cnt_to=DelayLen - bram_latency - 1  operation=Up  start_count=0  cnt_by_val=1  arith_type=Unsigned  n_bits=4  bin_pt=0  load_pin=off  rst=off  en=off  explicit_period=on  period=1  use_behavioral_HDL=on  implementation=Fabric  use_rpm=off  dbl_ovrd=off  block_type=counter
  ram : xbsIndex_r4/Single Port RAM  depth=16  initVector=0  distributed_mem=Block RAM  write_mode=Read Before Write  rst=off  init_reg=0  en=off  optimize_latency=off  latency=bram_latency  optimize=Area  dbl_ovrd=off  simulation_type=fast_sim  block_type=spram
  dout : Outport  VectorParamsAs1DForOutWhenUnconnected=off
  wires:
  counter/1 -> ram/1
  din/1 -> ram/2
  constant/1 -> ram/3
  ram/1 -> dout/1

== system rfsoc4x2_ospfb_128/pfb_fir_real10/pol1_in1_first_tap3/delay_bram ==
  din : Inport
  constant : xbsIndex_r4/Constant  const=1  gui_display_data_type=Fixed-point  arith_type=Boolean  n_bits=16  bin_pt=14  preci_type=Single  exp_width=8  frac_width=24  explicit_period=on  period=1  equ=P=C  opselect=C  inp2=PCIN>>17  opr=+  inp1=P  carry=CIN  dbl_ovrd=off  block_type=constant
  counter : xbsIndex_r4/Counter  cnt_type=Count Limited  cnt_to=DelayLen - bram_latency - 1  operation=Up  start_count=0  cnt_by_val=1  arith_type=Unsigned  n_bits=4  bin_pt=0  load_pin=off  rst=off  en=off  explicit_period=on  period=1  use_behavioral_HDL=on  implementation=Fabric  use_rpm=off  dbl_ovrd=off  block_type=counter
  ram : xbsIndex_r4/Single Port RAM  depth=16  initVector=0  distributed_mem=Block RAM  write_mode=Read Before Write  rst=off  init_reg=0  en=off  optimize_latency=off  latency=bram_latency  optimize=Area  dbl_ovrd=off  simulation_type=fast_sim  block_type=spram
  dout : Outport  VectorParamsAs1DForOutWhenUnconnected=off
  wires:
  counter/1 -> ram/1
  din/1 -> ram/2
  constant/1 -> ram/3
  ram/1 -> dout/1
